simulink model "pid_analog_fast"  (R2024b)
settings: Solver=ode4  StartTime=0.0  StopTime=10.0  FixedStep=pcb.sim_dt  RelTol=1e-3
PostLoadFcn:
  | pbdir_ = fileparts(get_param('pid_analog_fast', 'FileName')); if ~exist('pcb', 'var'), run(fullfile(pbdir_, 'pid_board_params.m')); end; if ~exist('CtrlIn', 'var'), run(fullfile(pbdir_, '..', 'common', 'quad_ctrl_buses.m')); end; clear pbdir_
values from neighbouring files (symbols this model uses):
  pcb = evalin('base', 'pcb')    [pid_analog_circuit_test.m]    (also in pid_board_bench_inputs.m; pid_board_params.m = struct(); pid_board_validate.m)
libraries: simulink x3
Description:
  | PID_Board rev B analog section, behavioural (fast) model. Ports: absolute node voltages, see ANALOG_INTERFACE.md. Parameters: pcb (pid_board_params.m).
settings Model: Creator=doubi  LastModifiedBy=doubi

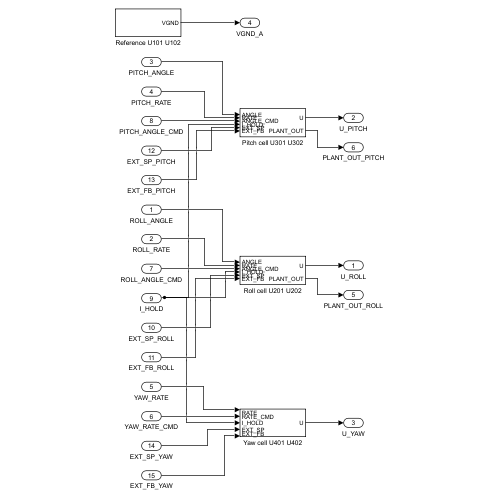
[thumbnail: Simulink's stored preview of the top-level diagram]
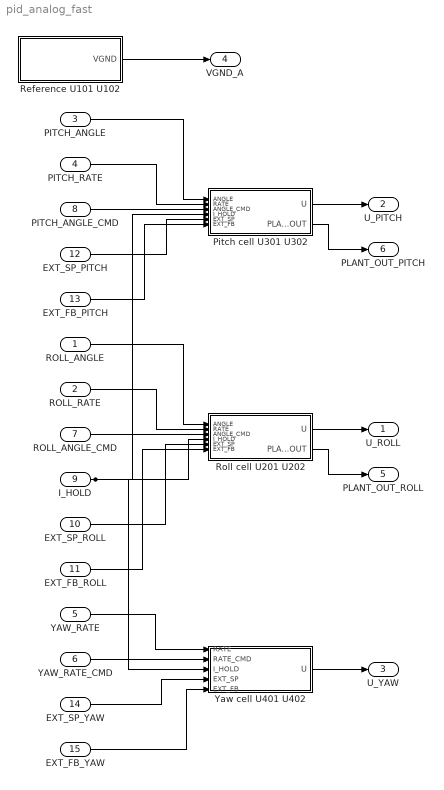
== system pid_analog_fast ==
  ROLL_ANGLE : Inport  OutDataTypeStr=double
  ROLL_RATE : Inport  Port=2  OutDataTypeStr=double
  PITCH_ANGLE : Inport  Port=3  OutDataTypeStr=double
  PITCH_RATE : Inport  Port=4  OutDataTypeStr=double
  YAW_RATE : Inport  Port=5  OutDataTypeStr=double
  YAW_RATE_CMD : Inport  Port=6  OutDataTypeStr=double
  ROLL_ANGLE_CMD : Inport  Port=7  OutDataTypeStr=double
  PITCH_ANGLE_CMD : Inport  Port=8  OutDataTypeStr=double
  I_HOLD : Inport  Port=9  OutDataTypeStr=double
  EXT_SP_ROLL : Inport  Port=10  OutDataTypeStr=double
  EXT_FB_ROLL : Inport  Port=11  OutDataTypeStr=double
  EXT_SP_PITCH : Inport  Port=12  OutDataTypeStr=double
  EXT_FB_PITCH : Inport  Port=13  OutDataTypeStr=double
  EXT_SP_YAW : Inport  Port=14  OutDataTypeStr=double
  EXT_FB_YAW : Inport  Port=15  OutDataTypeStr=double
  Pitch cell U301 U302 : Subsystem  mask{brd=pcb, ax=pcb.pitch}
      mask init:
      | vg = brd.ref.ideal*brd.VG + (1 - brd.ref.ideal)*brd.ref.V_tl431*brd.ref.RV_set_wiper_gnd/brd.ref.RV_set;
      | rlo = brd.V_rail_lo + brd.VG - vg;
      | rhi = brd.V_rail_hi + brd.VG - vg;
      | % Stage 1 diff amp: SP leg gain depends on both source impedances (jumper dependent)
      | jpsp = ax.JP_SP; jpfb = ax.JP_FB;
      | rsp = (jpsp == 1)*ax.R_src_sp; rfb = (jpfb == 1)*ax.R_src_fb;
      | gsp = ax.R_dsp_ref/(ax.R_dsp_in + rsp + ax.R_dsp_ref)*(1 + ax.R_dfb_f/(ax.R_dfb_in + rfb));
      | gfb = ax.R_dfb_f/(ax.R_dfb_in + ax.R_src_fb);
      | gfbx = ax.R_dfb_f/ax.R_dfb_in;
      | tauInv = brd.dac.tau_inv_leg; tauNi = brd.dac.tau_ni_leg;
      | % Stage 2 P, 3 leaky I + clamp + CD4066, 4 band-limited D
      | Kp = (ax.R_P_fixed + ax.RV_P)/ax.R_P_in;
      | kI = 1/((ax.R_I_fixed + ax.RV_I)*ax.CI);
      | wL = 1/(ax.RL*ax.CI);
      | wH = 1/(brd.ihold.R_on*ax.CI);
      | Vcl = min([ax.V_iclamp, rhi, -rlo]);
      | Rd = ax.Rd_fixed + ax.RV_D;
      | numD = [-Rd*ax.Cd 0];
      | denD = conv([ax.Rs*ax.Cd 1], [Rd*ax.Cf 1]);
      | enP = ax.en_P; enI = ax.en_I; enD = ax.en_D;
      | Vth = brd.VDD/2;
      | % Stage 6 angle diff (swapped legs), 7 angle P, 8 bench plant
      | gac = ax.R_a_f/(ax.R_acmd_in + ax.R_src_ang);
      | gam = ax.R_a_ref/(ax.R_ameas_in + ax.R_src_ang + ax.R_a_ref)*(1 + ax.R_a_f/(ax.R_acmd_in + ax.R_src_ang));
      | Go = (ax.R_A_fixed + ax.RV_A)/ax.R_A_in;
      | kPl = 1/(ax.R_plant*ax.C_plant);
  Reference U101 U102 : Subsystem  mask{brd=pcb}
      mask init:
      | vg = brd.ref.ideal*brd.VG + (1 - brd.ref.ideal)*brd.ref.V_tl431*brd.ref.RV_set_wiper_gnd/brd.ref.RV_set;
      | rlo = brd.V_rail_lo + brd.VG - vg;
      | rhi = brd.V_rail_hi + brd.VG - vg;
  Roll cell U201 U202 : Subsystem  mask{brd=pcb, ax=pcb.roll}
      mask init: same as pid_analog_fast/Pitch cell U301 U302
  Yaw cell U401 U402 : Subsystem  mask{brd=pcb, ax=pcb.yaw}
      mask init:
      | vg = brd.ref.ideal*brd.VG + (1 - brd.ref.ideal)*brd.ref.V_tl431*brd.ref.RV_set_wiper_gnd/brd.ref.RV_set;
      | rlo = brd.V_rail_lo + brd.VG - vg;
      | rhi = brd.V_rail_hi + brd.VG - vg;
      | % Stage 1 diff amp: SP leg gain depends on both source impedances (jumper dependent)
      | jpsp = ax.JP_SP; jpfb = ax.JP_FB;
      | rsp = (jpsp == 1)*ax.R_src_sp; rfb = (jpfb == 1)*ax.R_src_fb;
      | gsp = ax.R_dsp_ref/(ax.R_dsp_in + rsp + ax.R_dsp_ref)*(1 + ax.R_dfb_f/(ax.R_dfb_in + rfb));
      | gfb = ax.R_dfb_f/(ax.R_dfb_in + ax.R_src_fb);
      | gfbx = ax.R_dfb_f/ax.R_dfb_in;
      | tauInv = brd.dac.tau_inv_leg; tauNi = brd.dac.tau_ni_leg;
      | % Stage 2 P, 3 leaky I + clamp + CD4066, 4 band-limited D
      | Kp = (ax.R_P_fixed + ax.RV_P)/ax.R_P_in;
      | kI = 1/((ax.R_I_fixed + ax.RV_I)*ax.CI);
      | wL = 1/(ax.RL*ax.CI);
      | wH = 1/(brd.ihold.R_on*ax.CI);
      | Vcl = min([ax.V_iclamp, rhi, -rlo]);
      | Rd = ax.Rd_fixed + ax.RV_D;
      | numD = [-Rd*ax.Cd 0];
      | denD = conv([ax.Rs*ax.Cd 1], [Rd*ax.Cf 1]);
      | enP = ax.en_P; enI = ax.en_I; enD = ax.en_D;
      | Vth = brd.VDD/2;
  U_ROLL : Outport
  U_PITCH : Outport  Port=2
  U_YAW : Outport  Port=3
  VGND_A : Outport  Port=4
  PLANT_OUT_ROLL : Outport  Port=5
  PLANT_OUT_PITCH : Outport  Port=6
  wires:
  PITCH_ANGLE/1 -> Pitch cell U301 U302/1(ANGLE)
  PITCH_RATE/1 -> Pitch cell U301 U302/2(RATE)
  ROLL_ANGLE/1 -> Roll cell U201 U202/1(ANGLE)
  ROLL_RATE/1 -> Roll cell U201 U202/2(RATE)
  Reference U101 U102/1(VGND) -> VGND_A/1
  YAW_RATE_CMD/1 -> Yaw cell U401 U402/2(RATE_CMD)
  YAW_RATE/1 -> Yaw cell U401 U402/1(RATE)
  ROLL_ANGLE_CMD/1 -> Roll cell U201 U202/3(ANGLE_CMD)
  PITCH_ANGLE_CMD/1 -> Pitch cell U301 U302/3(ANGLE_CMD)
  EXT_FB_ROLL/1 -> Roll cell U201 U202/6(EXT_FB)
  EXT_SP_ROLL/1 -> Roll cell U201 U202/5(EXT_SP)
  I_HOLD/1 -> Pitch cell U301 U302/4(I_HOLD), Yaw cell U401 U402/3(I_HOLD), Roll cell U201 U202/4(I_HOLD)
  EXT_SP_PITCH/1 -> Pitch cell U301 U302/5(EXT_SP)
  EXT_FB_YAW/1 -> Yaw cell U401 U402/5(EXT_FB)
  EXT_SP_YAW/1 -> Yaw cell U401 U402/4(EXT_SP)
  EXT_FB_PITCH/1 -> Pitch cell U301 U302/6(EXT_FB)
  Pitch cell U301 U302/1(U) -> U_PITCH/1
  Pitch cell U301 U302/2(PLANT_OUT) -> PLANT_OUT_PITCH/1
  Roll cell U201 U202/1(U) -> U_ROLL/1
  Roll cell U201 U202/2(PLANT_OUT) -> PLANT_OUT_ROLL/1
  Yaw cell U401 U402/1(U) -> U_YAW/1

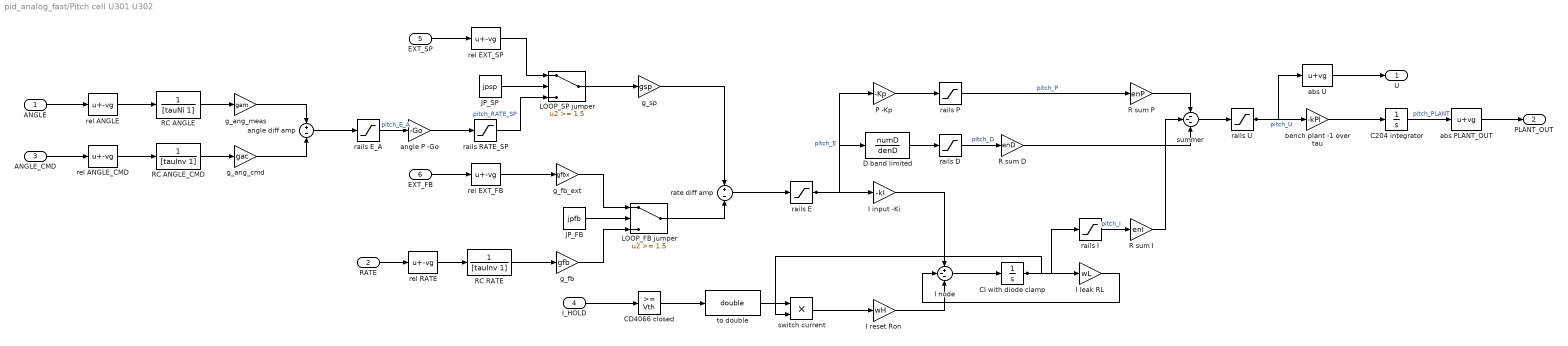
== system pid_analog_fast/Pitch cell U301 U302 ==
  ANGLE : Inport
  RATE : Inport  Port=2
  ANGLE_CMD : Inport  Port=3
  I_HOLD : Inport  Port=4
  EXT_SP : Inport  Port=5
  EXT_FB : Inport  Port=6
  C204 integrator : Integrator  LimitOutput=on  UpperSaturationLimit=rhi  LowerSaturationLimit=rlo
  CD4066 closed : simulink/Logic and Bit Operations/Compare To Constant  relop=>=  const=Vth  OutDataTypeStr=boolean
  CI with diode clamp : Integrator  LimitOutput=on  UpperSaturationLimit=Vcl  LowerSaturationLimit=-Vcl
  D band limited : TransferFcn  Numerator=numD  Denominator=denD
  I input -Ki : Gain  Gain=-kI
  I leak RL : Gain  Gain=wL
  I node : Sum  Inputs=+--
  I reset Ron : Gain  Gain=wH
  JP_FB : Constant  Value=jpfb
  JP_SP : Constant  Value=jpsp
  LOOP_FB jumper : Switch  Threshold=1.5  SaturateOnIntegerOverflow=off  InputSameDT=off
  LOOP_SP jumper : Switch  Threshold=1.5  SaturateOnIntegerOverflow=off  InputSameDT=off
  P -Kp : Gain  Gain=-Kp
  R sum D : Gain  Gain=enD
  R sum I : Gain  Gain=enI
  R sum P : Gain  Gain=enP
  RC ANGLE : TransferFcn  Numerator=1  Denominator=[tauNi 1]
  RC ANGLE_CMD : TransferFcn  Numerator=1  Denominator=[tauInv 1]
  RC RATE : TransferFcn  Numerator=1  Denominator=[tauInv 1]
  abs PLANT_OUT : Bias  Bias=vg  SaturateOnIntegerOverflow=off
  abs U : Bias  Bias=vg  SaturateOnIntegerOverflow=off
  angle P -Go : Gain  Gain=-Go
  angle diff amp : Sum  Inputs=+-
  bench plant -1 over tau : Gain  Gain=-kPl
  g_ang_cmd : Gain  Gain=gac
  g_ang_meas : Gain  Gain=gam
  g_fb : Gain  Gain=gfb
  g_fb_ext : Gain  Gain=gfbx
  g_sp : Gain  Gain=gsp
  rails D : Saturate  UpperLimit=rhi  LowerLimit=rlo
  rails E : Saturate  UpperLimit=rhi  LowerLimit=rlo
  rails E_A : Saturate  UpperLimit=rhi  LowerLimit=rlo
  rails I : Saturate  UpperLimit=rhi  LowerLimit=rlo
  rails P : Saturate  UpperLimit=rhi  LowerLimit=rlo
  rails RATE_SP : Saturate  UpperLimit=rhi  LowerLimit=rlo
  rails U : Saturate  UpperLimit=rhi  LowerLimit=rlo
  rate diff amp : Sum  Inputs=+-
  rel ANGLE : Bias  Bias=-vg  SaturateOnIntegerOverflow=off
  rel ANGLE_CMD : Bias  Bias=-vg  SaturateOnIntegerOverflow=off
  rel EXT_FB : Bias  Bias=-vg  SaturateOnIntegerOverflow=off
  rel EXT_SP : Bias  Bias=-vg  SaturateOnIntegerOverflow=off
  rel RATE : Bias  Bias=-vg  SaturateOnIntegerOverflow=off
  summer : Sum  Inputs=---
  switch current : Product
  to double : DataTypeConversion  OutDataTypeStr=double  SaturateOnIntegerOverflow=off  RndMeth=Floor
  U : Outport
  PLANT_OUT : Outport  Port=2
  wires:
  ANGLE/1 -> rel ANGLE/1
  ANGLE_CMD/1 -> rel ANGLE_CMD/1
  g_fb_ext/1 -> LOOP_FB jumper/1
  g_ang_meas/1 -> angle diff amp/1
  RC ANGLE_CMD/1 -> g_ang_cmd/1
  RC ANGLE/1 -> g_ang_meas/1
  rel ANGLE_CMD/1 -> RC ANGLE_CMD/1
  JP_FB/1 -> LOOP_FB jumper/2
  rel ANGLE/1 -> RC ANGLE/1
  g_ang_cmd/1 -> angle diff amp/2
  angle diff amp/1 -> rails E_A/1
  rails E_A/1 -> angle P -Go/1  "pitch_E_A"
  RATE/1 -> rel RATE/1
  RC RATE/1 -> g_fb/1
  EXT_SP/1 -> rel EXT_SP/1
  angle P -Go/1 -> rails RATE_SP/1
  g_fb/1 -> LOOP_FB jumper/3
  EXT_FB/1 -> rel EXT_FB/1
  I_HOLD/1 -> CD4066 closed/1
  rel RATE/1 -> RC RATE/1
  rel EXT_SP/1 -> LOOP_SP jumper/1
  rails RATE_SP/1 -> LOOP_SP jumper/3  "pitch_RATE_SP"
  JP_SP/1 -> LOOP_SP jumper/2
  rel EXT_FB/1 -> g_fb_ext/1
  rails P/1 -> R sum P/1  "pitch_P"
  LOOP_SP jumper/1 -> g_sp/1
  g_sp/1 -> rate diff amp/1
  LOOP_FB jumper/1 -> rate diff amp/2
  I input -Ki/1 -> I node/1
  CD4066 closed/1 -> to double/1
  rate diff amp/1 -> rails E/1
  to double/1 -> switch current/1
  rails E/1 -> I input -Ki/1, D band limited/1, P -Kp/1  "pitch_E"
  switch current/1 -> I reset Ron/1
  P -Kp/1 -> rails P/1
  I node/1 -> CI with diode clamp/1
  D band limited/1 -> rails D/1
  I reset Ron/1 -> I node/3
  rails D/1 -> R sum D/1  "pitch_D"
  rails U/1 -> bench plant -1 over tau/1, abs U/1  "pitch_U"
  R sum D/1 -> summer/3
  CI with diode clamp/1 -> I leak RL/1, switch current/2, rails I/1
  rails I/1 -> R sum I/1  "pitch_I"
  I leak RL/1 -> I node/2
  R sum P/1 -> summer/1
  R sum I/1 -> summer/2
  summer/1 -> rails U/1
  abs U/1 -> U/1
  bench plant -1 over tau/1 -> C204 integrator/1
  C204 integrator/1 -> abs PLANT_OUT/1  "pitch_PLANT"
  abs PLANT_OUT/1 -> PLANT_OUT/1

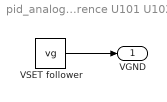
== system pid_analog_fast/Reference U101 U102 ==
  VSET follower : Constant  Value=vg  SampleTime=0
  VGND : Outport
  wires:
  VSET follower/1 -> VGND/1

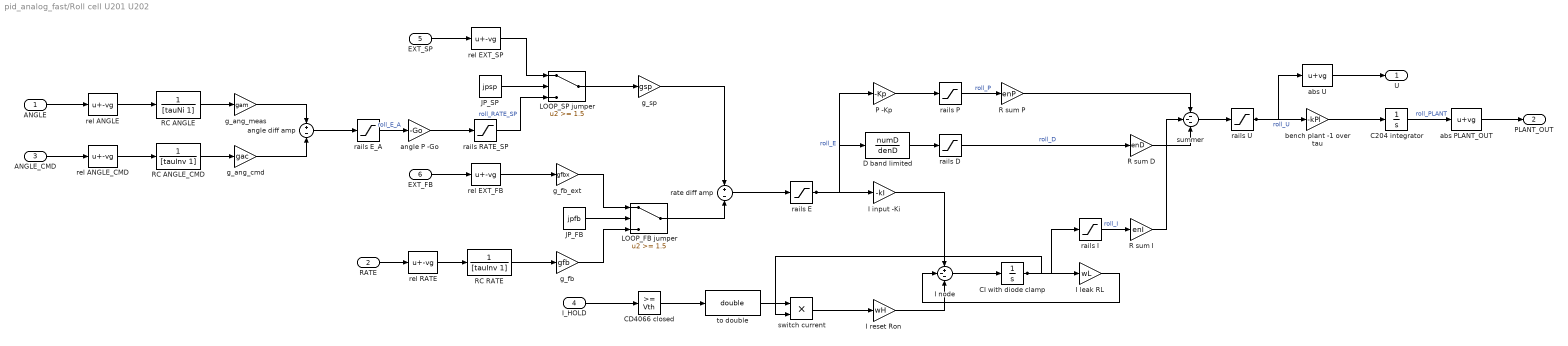
== system pid_analog_fast/Roll cell U201 U202 ==
  ANGLE : Inport
  RATE : Inport  Port=2
  ANGLE_CMD : Inport  Port=3
  I_HOLD : Inport  Port=4
  EXT_SP : Inport  Port=5
  EXT_FB : Inport  Port=6
  C204 integrator : Integrator  LimitOutput=on  UpperSaturationLimit=rhi  LowerSaturationLimit=rlo
  CD4066 closed : simulink/Logic and Bit Operations/Compare To Constant  relop=>=  const=Vth  OutDataTypeStr=boolean
  CI with diode clamp : Integrator  LimitOutput=on  UpperSaturationLimit=Vcl  LowerSaturationLimit=-Vcl
  D band limited : TransferFcn  Numerator=numD  Denominator=denD
  I input -Ki : Gain  Gain=-kI
  I leak RL : Gain  Gain=wL
  I node : Sum  Inputs=+--
  I reset Ron : Gain  Gain=wH
  JP_FB : Constant  Value=jpfb
  JP_SP : Constant  Value=jpsp
  LOOP_FB jumper : Switch  Threshold=1.5  SaturateOnIntegerOverflow=off  InputSameDT=off
  LOOP_SP jumper : Switch  Threshold=1.5  SaturateOnIntegerOverflow=off  InputSameDT=off
  P -Kp : Gain  Gain=-Kp
  R sum D : Gain  Gain=enD
  R sum I : Gain  Gain=enI
  R sum P : Gain  Gain=enP
  RC ANGLE : TransferFcn  Numerator=1  Denominator=[tauNi 1]
  RC ANGLE_CMD : TransferFcn  Numerator=1  Denominator=[tauInv 1]
  RC RATE : TransferFcn  Numerator=1  Denominator=[tauInv 1]
  abs PLANT_OUT : Bias  Bias=vg  SaturateOnIntegerOverflow=off
  abs U : Bias  Bias=vg  SaturateOnIntegerOverflow=off
  angle P -Go : Gain  Gain=-Go
  angle diff amp : Sum  Inputs=+-
  bench plant -1 over tau : Gain  Gain=-kPl
  g_ang_cmd : Gain  Gain=gac
  g_ang_meas : Gain  Gain=gam
  g_fb : Gain  Gain=gfb
  g_fb_ext : Gain  Gain=gfbx
  g_sp : Gain  Gain=gsp
  rails D : Saturate  UpperLimit=rhi  LowerLimit=rlo
  rails E : Saturate  UpperLimit=rhi  LowerLimit=rlo
  rails E_A : Saturate  UpperLimit=rhi  LowerLimit=rlo
  rails I : Saturate  UpperLimit=rhi  LowerLimit=rlo
  rails P : Saturate  UpperLimit=rhi  LowerLimit=rlo
  rails RATE_SP : Saturate  UpperLimit=rhi  LowerLimit=rlo
  rails U : Saturate  UpperLimit=rhi  LowerLimit=rlo
  rate diff amp : Sum  Inputs=+-
  rel ANGLE : Bias  Bias=-vg  SaturateOnIntegerOverflow=off
  rel ANGLE_CMD : Bias  Bias=-vg  SaturateOnIntegerOverflow=off
  rel EXT_FB : Bias  Bias=-vg  SaturateOnIntegerOverflow=off
  rel EXT_SP : Bias  Bias=-vg  SaturateOnIntegerOverflow=off
  rel RATE : Bias  Bias=-vg  SaturateOnIntegerOverflow=off
  summer : Sum  Inputs=---
  switch current : Product
  to double : DataTypeConversion  OutDataTypeStr=double  SaturateOnIntegerOverflow=off  RndMeth=Floor
  U : Outport
  PLANT_OUT : Outport  Port=2
  wires:
  g_sp/1 -> rate diff amp/1
  ANGLE/1 -> rel ANGLE/1
  rails RATE_SP/1 -> LOOP_SP jumper/3  "roll_RATE_SP"
  ANGLE_CMD/1 -> rel ANGLE_CMD/1
  C204 integrator/1 -> abs PLANT_OUT/1  "roll_PLANT"
  RC ANGLE/1 -> g_ang_meas/1
  rel ANGLE/1 -> RC ANGLE/1
  g_ang_cmd/1 -> angle diff amp/2
  g_ang_meas/1 -> angle diff amp/1
  RC ANGLE_CMD/1 -> g_ang_cmd/1
  rel ANGLE_CMD/1 -> RC ANGLE_CMD/1
  angle diff amp/1 -> rails E_A/1
  rails E_A/1 -> angle P -Go/1  "roll_E_A"
  P -Kp/1 -> rails P/1
  RATE/1 -> rel RATE/1
  rails E/1 -> P -Kp/1, I input -Ki/1, D band limited/1  "roll_E"
  EXT_SP/1 -> rel EXT_SP/1
  angle P -Go/1 -> rails RATE_SP/1
  LOOP_SP jumper/1 -> g_sp/1
  EXT_FB/1 -> rel EXT_FB/1
  rel RATE/1 -> RC RATE/1
  rel EXT_SP/1 -> LOOP_SP jumper/1
  rate diff amp/1 -> rails E/1
  JP_SP/1 -> LOOP_SP jumper/2
  summer/1 -> rails U/1
  rel EXT_FB/1 -> g_fb_ext/1
  CI with diode clamp/1 -> switch current/2, rails I/1, I leak RL/1
  RC RATE/1 -> g_fb/1
  g_fb_ext/1 -> LOOP_FB jumper/1
  R sum P/1 -> summer/1
  D band limited/1 -> rails D/1
  JP_FB/1 -> LOOP_FB jumper/2
  g_fb/1 -> LOOP_FB jumper/3
  I_HOLD/1 -> CD4066 closed/1
  LOOP_FB jumper/1 -> rate diff amp/2
  CD4066 closed/1 -> to double/1
  to double/1 -> switch current/1
  switch current/1 -> I reset Ron/1
  I input -Ki/1 -> I node/1
  I reset Ron/1 -> I node/3
  I leak RL/1 -> I node/2
  rails P/1 -> R sum P/1  "roll_P"
  R sum I/1 -> summer/2
  rails D/1 -> R sum D/1  "roll_D"
  I node/1 -> CI with diode clamp/1
  rails I/1 -> R sum I/1  "roll_I"
  rails U/1 -> abs U/1, bench plant -1 over tau/1  "roll_U"
  R sum D/1 -> summer/3
  abs U/1 -> U/1
  bench plant -1 over tau/1 -> C204 integrator/1
  abs PLANT_OUT/1 -> PLANT_OUT/1

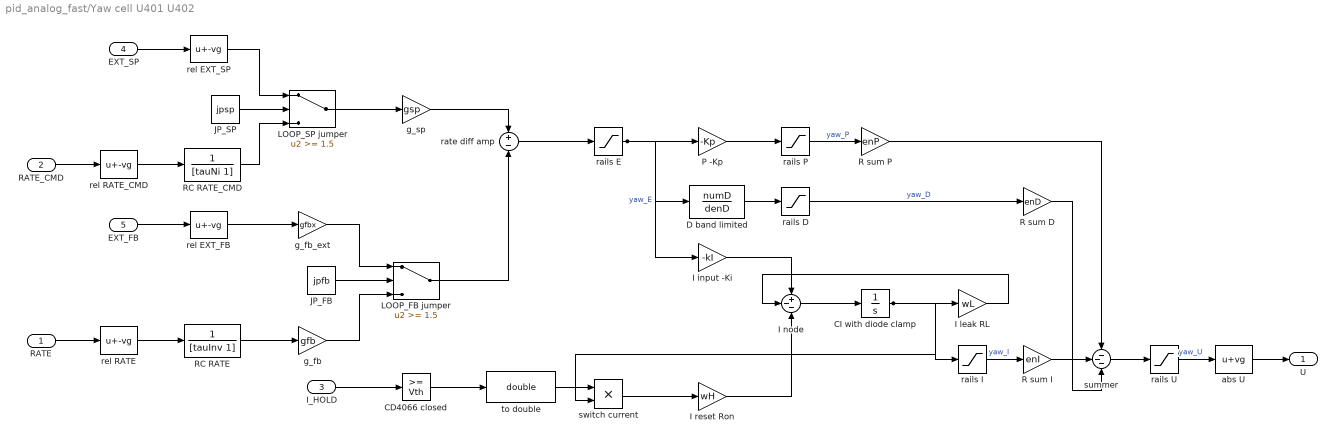
== system pid_analog_fast/Yaw cell U401 U402 ==
  RATE : Inport
  RATE_CMD : Inport  Port=2
  I_HOLD : Inport  Port=3
  EXT_SP : Inport  Port=4
  EXT_FB : Inport  Port=5
  CD4066 closed : simulink/Logic and Bit Operations/Compare To Constant  relop=>=  const=Vth  OutDataTypeStr=boolean
  CI with diode clamp : Integrator  LimitOutput=on  UpperSaturationLimit=Vcl  LowerSaturationLimit=-Vcl
  D band limited : TransferFcn  Numerator=numD  Denominator=denD
  I input -Ki : Gain  Gain=-kI
  I leak RL : Gain  Gain=wL
  I node : Sum  Inputs=+--
  I reset Ron : Gain  Gain=wH
  JP_FB : Constant  Value=jpfb
  JP_SP : Constant  Value=jpsp
  LOOP_FB jumper : Switch  Threshold=1.5  SaturateOnIntegerOverflow=off  InputSameDT=off
  LOOP_SP jumper : Switch  Threshold=1.5  SaturateOnIntegerOverflow=off  InputSameDT=off
  P -Kp : Gain  Gain=-Kp
  R sum D : Gain  Gain=enD
  R sum I : Gain  Gain=enI
  R sum P : Gain  Gain=enP
  RC RATE : TransferFcn  Numerator=1  Denominator=[tauInv 1]
  RC RATE_CMD : TransferFcn  Numerator=1  Denominator=[tauNi 1]
  abs U : Bias  Bias=vg  SaturateOnIntegerOverflow=off
  g_fb : Gain  Gain=gfb
  g_fb_ext : Gain  Gain=gfbx
  g_sp : Gain  Gain=gsp
  rails D : Saturate  UpperLimit=rhi  LowerLimit=rlo
  rails E : Saturate  UpperLimit=rhi  LowerLimit=rlo
  rails I : Saturate  UpperLimit=rhi  LowerLimit=rlo
  rails P : Saturate  UpperLimit=rhi  LowerLimit=rlo
  rails U : Saturate  UpperLimit=rhi  LowerLimit=rlo
  rate diff amp : Sum  Inputs=+-
  rel EXT_FB : Bias  Bias=-vg  SaturateOnIntegerOverflow=off
  rel EXT_SP : Bias  Bias=-vg  SaturateOnIntegerOverflow=off
  rel RATE : Bias  Bias=-vg  SaturateOnIntegerOverflow=off
  rel RATE_CMD : Bias  Bias=-vg  SaturateOnIntegerOverflow=off
  summer : Sum  Inputs=---
  switch current : Product
  to double : DataTypeConversion  OutDataTypeStr=double  SaturateOnIntegerOverflow=off  RndMeth=Floor
  U : Outport
  wires:
  EXT_FB/1 -> rel EXT_FB/1
  EXT_SP/1 -> rel EXT_SP/1
  RATE/1 -> rel RATE/1
  RATE_CMD/1 -> rel RATE_CMD/1
  rel RATE/1 -> RC RATE/1
  g_fb/1 -> LOOP_FB jumper/3
  JP_FB/1 -> LOOP_FB jumper/2
  rel RATE_CMD/1 -> RC RATE_CMD/1
  rate diff amp/1 -> rails E/1
  JP_SP/1 -> LOOP_SP jumper/2
  rel EXT_SP/1 -> LOOP_SP jumper/1
  RC RATE_CMD/1 -> LOOP_SP jumper/3
  rel EXT_FB/1 -> g_fb_ext/1
  LOOP_FB jumper/1 -> rate diff amp/2
  RC RATE/1 -> g_fb/1
  I leak RL/1 -> I node/2
  LOOP_SP jumper/1 -> g_sp/1
  g_fb_ext/1 -> LOOP_FB jumper/1
  I_HOLD/1 -> CD4066 closed/1
  g_sp/1 -> rate diff amp/1
  I input -Ki/1 -> I node/1
  CD4066 closed/1 -> to double/1
  to double/1 -> switch current/1
  rails E/1 -> P -Kp/1, I input -Ki/1, D band limited/1  "yaw_E"
  switch current/1 -> I reset Ron/1
  P -Kp/1 -> rails P/1
  R sum P/1 -> summer/1
  I node/1 -> CI with diode clamp/1
  D band limited/1 -> rails D/1
  I reset Ron/1 -> I node/3
  rails P/1 -> R sum P/1  "yaw_P"
  rails D/1 -> R sum D/1  "yaw_D"
  CI with diode clamp/1 -> I leak RL/1, rails I/1, switch current/2
  rails I/1 -> R sum I/1  "yaw_I"
  R sum D/1 -> summer/3
  R sum I/1 -> summer/2
  summer/1 -> rails U/1
  rails U/1 -> abs U/1  "yaw_U"
  abs U/1 -> U/1
